simulink model "TestModel"  (R2026b)
settings: Solver=FixedStepDiscrete  StopTime=inf  FixedStep=0.1
values from neighbouring files (symbols this model uses):
  inv_tau1 = 1 / tau1    (= 1)    [TestModelScript.m]
  inv_tau2 = 1 / tau2    (= 0.0666666666667)    [TestModelScript.m]
  inv_tau3 = 1 / tau3    (= 0.01)    [TestModelScript.m]
  OCV_Chg_Table = [ ... (first row only)    [TestModelScript.m]
  OCV_Dis_Table = [ ... (first row only)    [TestModelScript.m]
  R0_Chg_Table = w_R0 .* DCIR_Chg_Table    [TestModelScript.m]
  R0_Dis_Table = w_R0 .* DCIR_Dis_Table    [TestModelScript.m]
  R1_Chg_Table = w_R1 .* DCIR_Chg_Table    [TestModelScript.m]
  R1_Dis_Table = w_R1 .* DCIR_Dis_Table    [TestModelScript.m]
  R2_Chg_Table = w_R2 .* DCIR_Chg_Table    [TestModelScript.m]
  R2_Dis_Table = w_R2 .* DCIR_Dis_Table    [TestModelScript.m]
  R3_Chg_Table = w_R3 .* DCIR_Chg_Table    [TestModelScript.m]
  R3_Dis_Table = w_R3 .* DCIR_Dis_Table    [TestModelScript.m]
  SOC_bp_dcir = 0:10:100    [TestModelScript.m]
  SOC_bp_ocv = 0:5:100    [TestModelScript.m]
  SOC_gain = -100 / Q_nom_As    (= -0.00578703703704)    [TestModelScript.m]
  SOC_Inv_Chg_Tbl = zeros(length(V_bp_inv), length(Temp_bp_ocv))    [TestModelScript.m]
  SOC_Inv_Dis_Tbl = zeros(length(V_bp_inv), length(Temp_bp_ocv))    [TestModelScript.m]
  Temp_bp_dcir = [-20, -10, 0, 10, 25, 45, 60]    [TestModelScript.m]
  Temp_bp_ocv = [-20, -10, 0, 10, 25, 45, 55]    [TestModelScript.m]
  Temp_default = 25.0    (= 25)    [TestModelScript.m]
  V_bp_inv = linspace(2.90, 4.16, 64)    [TestModelScript.m]
undefined symbols (not defined in the file or in its folder): Active_DisChrg_E, Charger_Mode_E, Charger_Mode_Req_E, CV_Mode_Timer_E, DiscIntNeverNeededParam, OBC_E, VDU_MACHINE_STS_E
libraries: simulink x9
settings Model: PauseTimes=420  Creator=hp  LastModifiedBy=hari.r

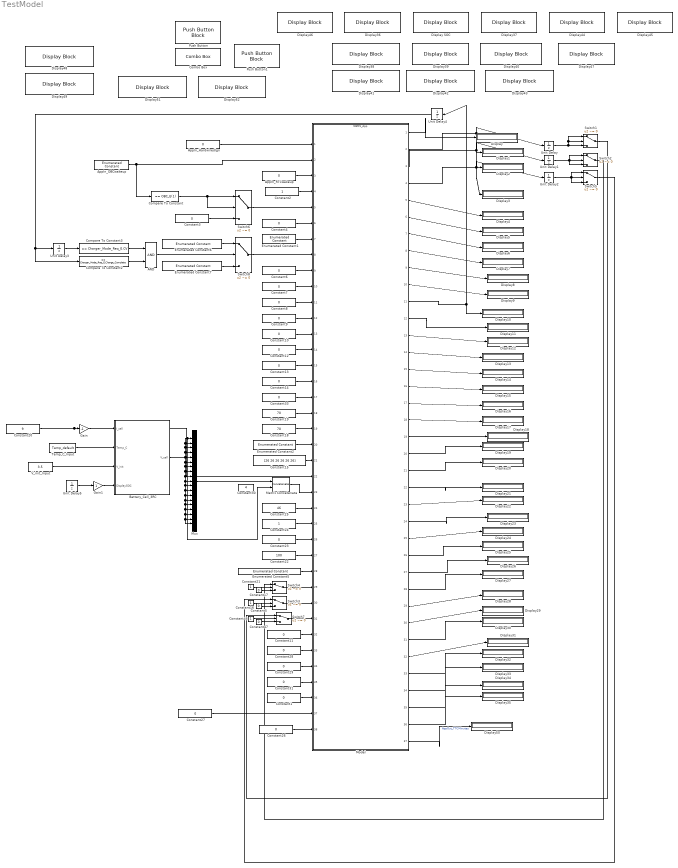
== system TestModel ==
  AND : Logic  AllPortsSameDT=off  OutDataTypeStr=boolean
  AppIn_HardwiredIgn : Constant  Value=0  OutDataTypeStr=boolean
  AppIn_OBCwakeup : simulink/Sources/Enumerated Constant  OutDataTypeStr=Enum: OBC_E  Value=OBC_E(1)  SampleTime=inf
  AppIn_RTCwakeup : Constant  Value=0  OutDataTypeStr=boolean
  Battery_Cell_3RC : Subsystem
  Combo Box : ComboBox  LabelPosition=Bottom  SelectedLabel=Wake_Up  UseEnumeratedDataType=on  EnumeratedDataType=OBC_E
  Compare To Constant : simulink/Logic and Bit Operations/Compare To Constant  relop===  const=OBC_E(1)  OutDataTypeStr=boolean
  Compare To Constant2 : simulink/Logic and Bit Operations/Compare To Constant  relop===  const=Charger_Mode_Req_E.Charge_Complete  OutDataTypeStr=boolean
  Compare To Constant3 : simulink/Logic and Bit Operations/Compare To Constant  relop===  const=Charger_Mode_Req_E.CV  OutDataTypeStr=boolean
  Constant{1,3..4,6..14,23,26..29,31,33} (19 alike) : Constant  Value=0  OutDataTypeStr=boolean
  Constant15 : Constant  Value=[26 26 26 26 26 26]  OutDataTypeStr=double
  Constant16 : Constant  OutDataTypeStr=Inherit: Inherit via back propagation
  Constant17 : Constant  Value=0  OutDataTypeStr=Inherit: Inherit via back propagation
  Constant18 : Constant  Value=70  OutDataTypeStr=double
  Constant19 : Constant  Value=70  OutDataTypeStr=double
  Constant2 : Constant  OutDataTypeStr=boolean
  Constant20 : Constant  Value=9  OutDataTypeStr=double
  Constant21 : Constant  OutDataTypeStr=Inherit: Inherit via back propagation
  Constant22 : Constant  Value=100  OutDataTypeStr=double
  Constant24 : Constant  OutDataTypeStr=double
  Constant25 : Constant  Value=46  OutDataTypeStr=double
  Constant30 : Constant  Value=4  OutDataTypeStr=Inherit: Inherit via back propagation
  Constant46 : Constant  OutDataTypeStr=Inherit: Inherit via back propagation
  Constant47 : Constant  Value=0  OutDataTypeStr=Inherit: Inherit via back propagation
  Constant5 : Constant  Value=0  OutDataTypeStr=Inherit: Inherit via back propagation
  Display{,1..35,50} (37 alike) : Display
  Display SOC : DisplayBlock  LabelPosition=Bottom  Transparency=1  GridColor=[0.502, 0.502, 0.502]
  Display{36..49,51..52} (16 alike) : DisplayBlock  LabelPosition=Bottom  Transparency=1  GridColor=[0.502, 0.502, 0.502]
  Enumerated Constant1 : simulink/Sources/Enumerated Constant  OutDataTypeStr=Enum: Charger_Mode_E  Value=Charger_Mode_E.OFF  SampleTime=inf
  Enumerated Constant2 : simulink/Sources/Enumerated Constant  OutDataTypeStr=Enum: Active_DisChrg_E  Value=Active_DisChrg_E.Inactive  SampleTime=inf
  Enumerated Constant5 : simulink/Sources/Enumerated Constant  OutDataTypeStr=Enum: VDU_MACHINE_STS_E  Value=VDU_MACHINE_STS_E.VDU_SLEEP  SampleTime=inf
  Enumerated Constant6 : simulink/Sources/Enumerated Constant  OutDataTypeStr=Enum: CV_Mode_Timer_E  Value=CV_Mode_Timer_E.Expired  SampleTime=inf
  Enumerated Constant7 : simulink/Sources/Enumerated Constant  OutDataTypeStr=Enum: CV_Mode_Timer_E  Value=CV_Mode_Timer_E.Off  SampleTime=inf
  Gain : Gain  Gain=-1
  Gain1 : Gain  OutDataTypeStr=double
  Matrix Concatenate : Concatenate  ConcatenateDimension=28
  Model : ModelReference  ModelNameDialog=NBMS_App.slx  SimulationMode=Normal  ModelReferenceVersion=1.0
  Mux : Mux  Inputs=19
  Push Button : PushButtonBlock  LabelPosition=Bottom  ButtonText=IgnKey  ButtonType=Latch  IconOnColor=[0.0, 0.39215686274509803, 0.0]  IconOffColor=[0.0, 1.0, 0.0]  OffValue=0.000000
  Push Button1 : PushButtonBlock  LabelPosition=Bottom  ButtonText=RTCWakeup  IconOnColor=[0.0, 0.39215686274509803, 0.0]  IconOffColor=[0.0, 1.0, 0.0]  OffValue=0.000000
  Switch{1..8} (8 alike) : Switch  Criteria=u2 ~= 0  SaturateOnIntegerOverflow=off  InputSameDT=off
  Temp_C_Input : Constant  Value=Temp_default
  Unit Delay : UnitDelay  SampleTime=-1
  Unit Delay1 : UnitDelay  SampleTime=-1
  Unit Delay2 : UnitDelay  SampleTime=-1
  Unit Delay3 : UnitDelay  InitialCondition=Charger_Mode_Req_E.Disabled  SampleTime=-1
  Unit Delay4 : UnitDelay  InitialCondition=Charger_Mode_Req_E.Disabled  SampleTime=-1
  Unit Delay5 : UnitDelay  InitialCondition=8  SampleTime=-1
  V_init_Input : Constant  Value=3.5
  wires:
  AppIn_HardwiredIgn/1 -> Model/1
  AppIn_OBCwakeup/1 -> Compare To Constant/1, Model/2
  AppIn_RTCwakeup/1 -> Model/3
  Constant4/1 -> Model/6
  Model/1 -> Display/1
  Model/2 -> Unit Delay/1, Display1/1
  Model/3 -> Unit Delay1/1, Display2/1
  Model/4 -> Display3/1, Unit Delay2/1
  Model/5 -> Display4/1
  Model/6 -> Display5/1
  Model/7 -> Display6/1
  Enumerated Constant1/1 -> Model/7
  Model/8 -> Display7/1
  Model/9 -> Display8/1
  Model/10 -> Display9/1
  Model/11 -> Unit Delay4/1, Display10/1
  Model/12 -> Display11/1
  Model/13 -> Display12/1
  Model/14 -> Display13/1
  Model/15 -> Display14/1
  Model/16 -> Display15/1
  Model/17 -> Display16/1
  Model/18 -> Display17/1
  Model/19 -> Display18/1
  Model/20 -> Display19/1
  Model/21 -> Display20/1
  Model/22 -> Display21/1
  Model/23 -> Display22/1
  Model/24 -> Display23/1
  Model/25 -> Display24/1
  Model/26 -> Display25/1
  Model/27 -> Display26/1
  Switch7/1 -> Model/31
  Constant47/1 -> Switch7/3
  Constant46/1 -> Switch7/2
  Unit Delay/1 -> Switch1/1, Switch1/2, Switch1/3
  Switch1/1 -> Switch7/1
  Unit Delay1/1 -> Switch2/1, Switch2/3, Switch2/2
  Switch3/1 -> Model/30
  Constant5/1 -> Switch3/3
  Constant16/1 -> Switch3/2
  Switch4/1 -> Model/29
  Constant17/1 -> Switch4/3
  Constant21/1 -> Switch4/2
  Unit Delay2/1 -> Switch5/1, Switch5/3, Switch5/2
  Enumerated Constant5/1 -> Model/28
  Constant22/1 -> Model/27
  Constant23/1 -> Model/26
  Constant24/1 -> Model/25
  Constant25/1 -> Model/24
  Battery_Cell_3RC/1(V_cell) -> Matrix Concatenate/2, Mux/1, Mux/2, Mux/3, Mux/4, Mux/18, Mux/19, Mux/17, Mux/16, Mux/15, Mux/14, Mux/13, Mux/12, Mux/11, Mux/10, Mux/9, Mux/8, Mux/7, Mux/6, Mux/5
  Mux/1 -> Matrix Concatenate/1
  Constant18/1 -> Model/19
  Constant15/1 -> Model/21
  Unit Delay3/1 -> Compare To Constant3/1
  Compare To Constant3/1 -> AND/1
  Compare To Constant2/1 -> AND/2
  AND/1 -> Switch8/2
  Enumerated Constant6/1 -> Switch8/1
  Enumerated Constant7/1 -> Switch8/3
  Switch8/1 -> Model/8
  Model/28 -> Display27/1
  Unit Delay4/1 -> Compare To Constant2/1, Unit Delay3/1
  Switch5/1 -> Switch3/1
  Switch2/1 -> Switch4/1
  Constant19/1 -> Model/18
  Constant14/1 -> Model/16
  Constant13/1 -> Model/15
  Constant12/1 -> Model/14
  Constant10/1 -> Model/13
  Constant9/1 -> Model/12
  Constant8/1 -> Model/11
  Constant7/1 -> Model/10
  Constant6/1 -> Model/9
  Model/29 -> Display28/1
  Model/30 -> Display29/1
  Model/31 -> Display30/1
  Constant11/1 -> Model/32
  Constant28/1 -> Model/33
  Constant29/1 -> Model/34
  Constant31/1 -> Model/35
  Matrix Concatenate/1 -> Model/23
  Constant33/1 -> Model/17
  Enumerated Constant2/1 -> Model/20
  Constant20/1 -> Model/22, Gain/1
  Model/32 -> Display31/1
  Model/33 -> Display32/1
  Model/34 -> Display33/1
  Model/35 -> Display34/1
  Model/36 -> Display35/1
  Constant3/1 -> Switch6/3
  Switch6/1 -> Model/5
  Constant2/1 -> Model/4
  Compare To Constant/1 -> Switch6/1, Switch6/2
  Constant1/1 -> Model/36
  V_init_Input/1 -> Battery_Cell_3RC/3(V_init)
  Temp_C_Input/1 -> Battery_Cell_3RC/2(Temp_C)
  Gain/1 -> Battery_Cell_3RC/1(I_cell)
  Unit Delay5/1 -> Gain1/1
  Gain1/1 -> Battery_Cell_3RC/4(DisplaySOC)
  Constant26/1 -> Model/38
  Constant27/1 -> Model/37
  Model/37 -> Display50/1  "AppOut_TTCMinutes"

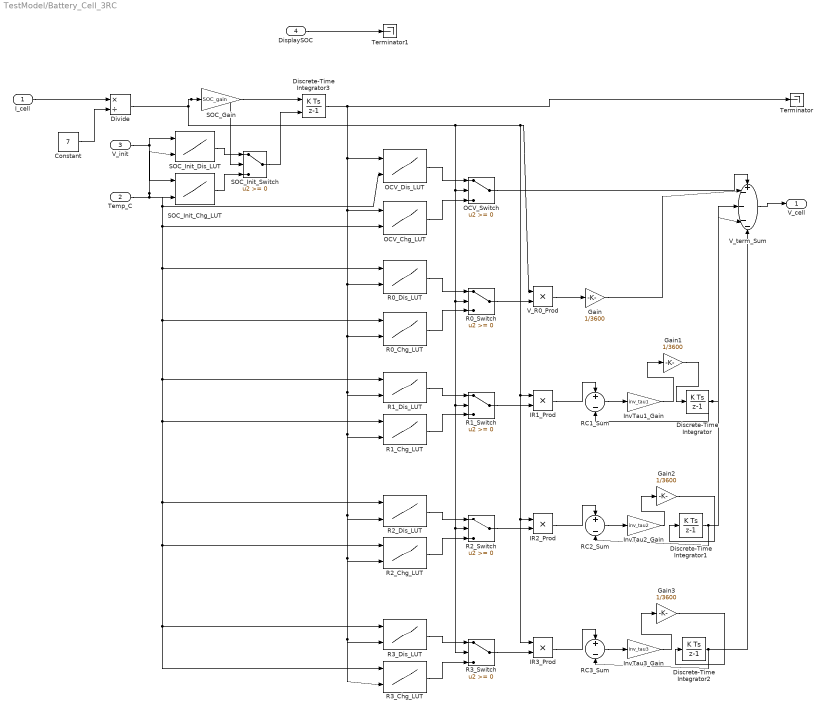
== system TestModel/Battery_Cell_3RC ==
  I_cell : Inport
  Temp_C : Inport  Port=2
  V_init : Inport  Port=3
  DisplaySOC : Inport  Port=4
  Constant : Constant  Value=7
  Discrete-Time Integrator : DiscreteIntegrator  SampleTime=-1  ICPrevOutput=DiscIntNeverNeededParam  ICPrevScaledInput=DiscIntNeverNeededParam
  Discrete-Time Integrator1 : DiscreteIntegrator  SampleTime=-1  ICPrevOutput=DiscIntNeverNeededParam  ICPrevScaledInput=DiscIntNeverNeededParam
  Discrete-Time Integrator2 : DiscreteIntegrator  SampleTime=-1  ICPrevOutput=DiscIntNeverNeededParam  ICPrevScaledInput=DiscIntNeverNeededParam
  Discrete-Time Integrator3 : DiscreteIntegrator  InitialConditionSource=external  SampleTime=-1  ICPrevOutput=DiscIntNeverNeededParam  ICPrevScaledInput=DiscIntNeverNeededParam
  Divide : Product  Inputs=*/
  Gain{,1..3} (4 alike) : Gain  Gain=1/3600
  IR1_Prod : Product
  IR2_Prod : Product
  IR3_Prod : Product
  InvTau1_Gain : Gain  Gain=inv_tau1
  InvTau2_Gain : Gain  Gain=inv_tau2
  InvTau3_Gain : Gain  Gain=inv_tau3
  OCV_Chg_LUT : Lookup_n-D  BreakpointsForDimension1=SOC_bp_ocv  BreakpointsForDimension2=Temp_bp_ocv  Table=OCV_Chg_Table  InternalRulePriority=Speed  RndMeth=Simplest
      settings: InputPortMap=u0,u1
  OCV_Dis_LUT : Lookup_n-D  BreakpointsForDimension1=SOC_bp_ocv  BreakpointsForDimension2=Temp_bp_ocv  Table=OCV_Dis_Table  InternalRulePriority=Speed  RndMeth=Simplest
      settings: InputPortMap=u0,u1
  OCV_Switch : Switch  SaturateOnIntegerOverflow=off  InputSameDT=off
  R0_Chg_LUT : Lookup_n-D  BreakpointsForDimension1=Temp_bp_dcir  BreakpointsForDimension2=SOC_bp_dcir  Table=R0_Chg_Table  InternalRulePriority=Speed  RndMeth=Simplest
      settings: InputPortMap=u0,u1
  R0_Dis_LUT : Lookup_n-D  BreakpointsForDimension1=Temp_bp_dcir  BreakpointsForDimension2=SOC_bp_dcir  Table=R0_Dis_Table  InternalRulePriority=Speed  RndMeth=Simplest
      settings: InputPortMap=u0,u1
  R0_Switch : Switch  SaturateOnIntegerOverflow=off  InputSameDT=off
  R1_Chg_LUT : Lookup_n-D  BreakpointsForDimension1=Temp_bp_dcir  BreakpointsForDimension2=SOC_bp_dcir  Table=R1_Chg_Table  InternalRulePriority=Speed  RndMeth=Simplest
      settings: InputPortMap=u0,u1
  R1_Dis_LUT : Lookup_n-D  BreakpointsForDimension1=Temp_bp_dcir  BreakpointsForDimension2=SOC_bp_dcir  Table=R1_Dis_Table  InternalRulePriority=Speed  RndMeth=Simplest
      settings: InputPortMap=u0,u1
  R1_Switch : Switch  SaturateOnIntegerOverflow=off  InputSameDT=off
  R2_Chg_LUT : Lookup_n-D  BreakpointsForDimension1=Temp_bp_dcir  BreakpointsForDimension2=SOC_bp_dcir  Table=R2_Chg_Table  InternalRulePriority=Speed  RndMeth=Simplest
      settings: InputPortMap=u0,u1
  R2_Dis_LUT : Lookup_n-D  BreakpointsForDimension1=Temp_bp_dcir  BreakpointsForDimension2=SOC_bp_dcir  Table=R2_Dis_Table  InternalRulePriority=Speed  RndMeth=Simplest
      settings: InputPortMap=u0,u1
  R2_Switch : Switch  SaturateOnIntegerOverflow=off  InputSameDT=off
  R3_Chg_LUT : Lookup_n-D  BreakpointsForDimension1=Temp_bp_dcir  BreakpointsForDimension2=SOC_bp_dcir  Table=R3_Chg_Table  InternalRulePriority=Speed  RndMeth=Simplest
      settings: InputPortMap=u0,u1
  R3_Dis_LUT : Lookup_n-D  BreakpointsForDimension1=Temp_bp_dcir  BreakpointsForDimension2=SOC_bp_dcir  Table=R3_Dis_Table  InternalRulePriority=Speed  RndMeth=Simplest
      settings: InputPortMap=u0,u1
  R3_Switch : Switch  SaturateOnIntegerOverflow=off  InputSameDT=off
  RC1_Sum : Sum  Inputs=+-
  RC2_Sum : Sum  Inputs=+-
  RC3_Sum : Sum  Inputs=+-
  SOC_Gain : Gain  Gain=SOC_gain
  SOC_Init_Chg_LUT : Lookup_n-D  BreakpointsForDimension1=V_bp_inv  BreakpointsForDimension2=Temp_bp_ocv  Table=SOC_Inv_Chg_Tbl  InternalRulePriority=Speed  RndMeth=Simplest
      settings: InputPortMap=u0,u1
  SOC_Init_Dis_LUT : Lookup_n-D  BreakpointsForDimension1=V_bp_inv  BreakpointsForDimension2=Temp_bp_ocv  Table=SOC_Inv_Dis_Tbl  InternalRulePriority=Speed  RndMeth=Simplest
      settings: InputPortMap=u0,u1
  SOC_Init_Switch : Switch  SaturateOnIntegerOverflow=off  InputSameDT=off
  Terminator : Terminator
  Terminator1 : Terminator
  V_R0_Prod : Product
  V_term_Sum : Sum  Inputs=+----
  V_cell : Outport
  wires:
  V_init/1 -> SOC_Init_Dis_LUT/1, SOC_Init_Chg_LUT/1
  Temp_C/1 -> R3_Dis_LUT/1, R3_Chg_LUT/1, R2_Chg_LUT/1, R2_Dis_LUT/1, R1_Chg_LUT/1, R1_Dis_LUT/1, R0_Chg_LUT/1, R0_Dis_LUT/1, OCV_Chg_LUT/2, OCV_Dis_LUT/2, SOC_Init_Dis_LUT/2, SOC_Init_Chg_LUT/2
  SOC_Init_Dis_LUT/1 -> SOC_Init_Switch/1
  Divide/1 -> SOC_Init_Switch/2, SOC_Gain/1, R2_Switch/2, R3_Switch/2, R1_Switch/2, R0_Switch/2, OCV_Switch/2, IR2_Prod/1, IR3_Prod/1, IR1_Prod/1, V_R0_Prod/1
  SOC_Init_Chg_LUT/1 -> SOC_Init_Switch/3
  SOC_Gain/1 -> Discrete-Time Integrator3/1
  SOC_Init_Switch/1 -> Discrete-Time Integrator3/2
  Discrete-Time Integrator3/1 -> Terminator/1, R3_Dis_LUT/2, R3_Chg_LUT/2, R2_Chg_LUT/2, R2_Dis_LUT/2, R1_Chg_LUT/2, R1_Dis_LUT/2, R0_Chg_LUT/2, R0_Dis_LUT/2, OCV_Chg_LUT/1, OCV_Dis_LUT/1
  OCV_Dis_LUT/1 -> OCV_Switch/1
  OCV_Chg_LUT/1 -> OCV_Switch/3
  R0_Dis_LUT/1 -> R0_Switch/1
  R0_Chg_LUT/1 -> R0_Switch/3
  R0_Switch/1 -> V_R0_Prod/2
  R1_Dis_LUT/1 -> R1_Switch/1
  R1_Chg_LUT/1 -> R1_Switch/3
  R1_Switch/1 -> IR1_Prod/2
  IR1_Prod/1 -> RC1_Sum/1
  Discrete-Time Integrator/1 -> RC1_Sum/2, V_term_Sum/3
  RC1_Sum/1 -> InvTau1_Gain/1
  InvTau1_Gain/1 -> Gain1/1
  R2_Dis_LUT/1 -> R2_Switch/1
  R2_Chg_LUT/1 -> R2_Switch/3
  R2_Switch/1 -> IR2_Prod/2
  IR2_Prod/1 -> RC2_Sum/1
  Discrete-Time Integrator1/1 -> V_term_Sum/4, RC2_Sum/2
  RC2_Sum/1 -> InvTau2_Gain/1
  InvTau2_Gain/1 -> Gain2/1
  R3_Dis_LUT/1 -> R3_Switch/1
  R3_Chg_LUT/1 -> R3_Switch/3
  R3_Switch/1 -> IR3_Prod/2
  IR3_Prod/1 -> RC3_Sum/1
  Discrete-Time Integrator2/1 -> V_term_Sum/5, RC3_Sum/2
  RC3_Sum/1 -> InvTau3_Gain/1
  InvTau3_Gain/1 -> Gain3/1
  OCV_Switch/1 -> V_term_Sum/1
  V_term_Sum/1 -> V_cell/1
  V_R0_Prod/1 -> Gain/1
  Gain1/1 -> Discrete-Time Integrator/1
  Gain2/1 -> Discrete-Time Integrator1/1
  Gain3/1 -> Discrete-Time Integrator2/1
  Gain/1 -> V_term_Sum/2
  DisplaySOC/1 -> Terminator1/1
  I_cell/1 -> Divide/1
  Constant/1 -> Divide/2
